simulink model "rfsoc4x2_ospfb_128"  (R2021a)
settings: Solver=VariableStepAuto  StartTime=0.0  StopTime=2048  RelTol=1e-3
undefined symbols (not defined in the file): pfb_coeff_gen_calc
libraries: xbsIndex_r4 x25898, casper_library_delays x113, casper_library_misc x68, xps_library x1
(part 6 of 221)

== system rfsoc4x2_ospfb_128/pipeline ==
  d : Inport
  Register0 : xbsIndex_r4/Register  init=0  rst=off  en=off  dbl_ovrd=off  block_type=register
      settings: block_version=11.4
  Register1 : xbsIndex_r4/Register  init=0  rst=off  en=off  dbl_ovrd=off  block_type=register
  q : Outport  VectorParamsAs1DForOutWhenUnconnected=off
  wires:
  Register0/1 -> Register1/1
  d/1 -> Register0/1
  Register1/1 -> q/1

== system rfsoc4x2_ospfb_128/pipeline1 ==
  d : Inport
  Register0 : xbsIndex_r4/Register  init=0  rst=off  en=off  dbl_ovrd=off  block_type=register
      settings: block_version=11.4
  Register1 : xbsIndex_r4/Register  init=0  rst=off  en=off  dbl_ovrd=off  block_type=register
  q : Outport  VectorParamsAs1DForOutWhenUnconnected=off
  wires:
  Register0/1 -> Register1/1
  d/1 -> Register0/1
  Register1/1 -> q/1

== system rfsoc4x2_ospfb_128/pipeline100 ==
  d : Inport
  Register0 : xbsIndex_r4/Register  init=0  rst=off  en=off  dbl_ovrd=off  block_type=register
      settings: block_version=11.4
  q : Outport  VectorParamsAs1DForOutWhenUnconnected=off
  wires:
  d/1 -> Register0/1
  Register0/1 -> q/1

== system rfsoc4x2_ospfb_128/pipeline101 ==
  d : Inport
  Register0 : xbsIndex_r4/Register  init=0  rst=off  en=off  dbl_ovrd=off  block_type=register
      settings: block_version=11.4
  q : Outport  VectorParamsAs1DForOutWhenUnconnected=off
  wires:
  d/1 -> Register0/1
  Register0/1 -> q/1

== system rfsoc4x2_ospfb_128/pipeline102 ==
  d : Inport
  Register0 : xbsIndex_r4/Register  init=0  rst=off  en=off  dbl_ovrd=off  block_type=register
      settings: block_version=11.4
  q : Outport  VectorParamsAs1DForOutWhenUnconnected=off
  wires:
  d/1 -> Register0/1
  Register0/1 -> q/1

== system rfsoc4x2_ospfb_128/pipeline103 ==
  d : Inport
  Register0 : xbsIndex_r4/Register  init=0  rst=off  en=off  dbl_ovrd=off  block_type=register
      settings: block_version=11.4
  q : Outport  VectorParamsAs1DForOutWhenUnconnected=off
  wires:
  d/1 -> Register0/1
  Register0/1 -> q/1

== system rfsoc4x2_ospfb_128/pipeline104 ==
  d : Inport
  Register0 : xbsIndex_r4/Register  init=0  rst=off  en=off  dbl_ovrd=off  block_type=register
      settings: block_version=11.4
  q : Outport  VectorParamsAs1DForOutWhenUnconnected=off
  wires:
  d/1 -> Register0/1
  Register0/1 -> q/1

== system rfsoc4x2_ospfb_128/pipeline105 ==
  d : Inport
  Register0 : xbsIndex_r4/Register  init=0  rst=off  en=off  dbl_ovrd=off  block_type=register
      settings: block_version=11.4
  q : Outport  VectorParamsAs1DForOutWhenUnconnected=off
  wires:
  d/1 -> Register0/1
  Register0/1 -> q/1

== system rfsoc4x2_ospfb_128/pipeline106 ==
  d : Inport
  Register0 : xbsIndex_r4/Register  init=0  rst=off  en=off  dbl_ovrd=off  block_type=register
      settings: block_version=11.4
  q : Outport  VectorParamsAs1DForOutWhenUnconnected=off
  wires:
  d/1 -> Register0/1
  Register0/1 -> q/1

== system rfsoc4x2_ospfb_128/pipeline2 ==
  d : Inport
  Register0 : xbsIndex_r4/Register  init=0  rst=off  en=off  dbl_ovrd=off  block_type=register
      settings: block_version=11.4
  Register1 : xbsIndex_r4/Register  init=0  rst=off  en=off  dbl_ovrd=off  block_type=register
  q : Outport  VectorParamsAs1DForOutWhenUnconnected=off
  wires:
  Register1/1 -> q/1
  d/1 -> Register0/1
  Register0/1 -> Register1/1

== system rfsoc4x2_ospfb_128/pipeline54 ==
  d : Inport
  Register0 : xbsIndex_r4/Register  init=0  rst=off  en=off  dbl_ovrd=off  block_type=register
      settings: block_version=11.4
  q : Outport  VectorParamsAs1DForOutWhenUnconnected=off
  wires:
  d/1 -> Register0/1
  Register0/1 -> q/1

== system rfsoc4x2_ospfb_128/pipeline55 ==
  d : Inport
  Register0 : xbsIndex_r4/Register  init=0  rst=off  en=off  dbl_ovrd=off  block_type=register
      settings: block_version=11.4
  q : Outport  VectorParamsAs1DForOutWhenUnconnected=off
  wires:
  d/1 -> Register0/1
  Register0/1 -> q/1

== system rfsoc4x2_ospfb_128/pipeline56 ==
  d : Inport
  Register0 : xbsIndex_r4/Register  init=0  rst=off  en=off  dbl_ovrd=off  block_type=register
      settings: block_version=11.4
  q : Outport  VectorParamsAs1DForOutWhenUnconnected=off
  wires:
  d/1 -> Register0/1
  Register0/1 -> q/1

== system rfsoc4x2_ospfb_128/pipeline57 ==
  d : Inport
  Register0 : xbsIndex_r4/Register  init=0  rst=off  en=off  dbl_ovrd=off  block_type=register
      settings: block_version=11.4
  q : Outport  VectorParamsAs1DForOutWhenUnconnected=off
  wires:
  d/1 -> Register0/1
  Register0/1 -> q/1

== system rfsoc4x2_ospfb_128/pipeline58 ==
  d : Inport
  Register0 : xbsIndex_r4/Register  init=0  rst=off  en=off  dbl_ovrd=off  block_type=register
      settings: block_version=11.4
  q : Outport  VectorParamsAs1DForOutWhenUnconnected=off
  wires:
  d/1 -> Register0/1
  Register0/1 -> q/1

== system rfsoc4x2_ospfb_128/pipeline60 ==
  d : Inport
  Register0 : xbsIndex_r4/Register  init=0  rst=off  en=off  dbl_ovrd=off  block_type=register
      settings: block_version=11.4
  q : Outport  VectorParamsAs1DForOutWhenUnconnected=off
  wires:
  d/1 -> Register0/1
  Register0/1 -> q/1

== system rfsoc4x2_ospfb_128/pipeline61 ==
  d : Inport
  Register0 : xbsIndex_r4/Register  init=0  rst=off  en=off  dbl_ovrd=off  block_type=register
      settings: block_version=11.4
  q : Outport  VectorParamsAs1DForOutWhenUnconnected=off
  wires:
  d/1 -> Register0/1
  Register0/1 -> q/1

== system rfsoc4x2_ospfb_128/pipeline62 ==
  d : Inport
  Register0 : xbsIndex_r4/Register  init=0  rst=off  en=off  dbl_ovrd=off  block_type=register
      settings: block_version=11.4
  q : Outport  VectorParamsAs1DForOutWhenUnconnected=off
  wires:
  d/1 -> Register0/1
  Register0/1 -> q/1

== system rfsoc4x2_ospfb_128/pipeline63 ==
  d : Inport
  Register0 : xbsIndex_r4/Register  init=0  rst=off  en=off  dbl_ovrd=off  block_type=register
      settings: block_version=11.4
  q : Outport  VectorParamsAs1DForOutWhenUnconnected=off
  wires:
  d/1 -> Register0/1
  Register0/1 -> q/1

== system rfsoc4x2_ospfb_128/pipeline64 ==
  d : Inport
  Register0 : xbsIndex_r4/Register  init=0  rst=off  en=off  dbl_ovrd=off  block_type=register
      settings: block_version=11.4
  q : Outport  VectorParamsAs1DForOutWhenUnconnected=off
  wires:
  d/1 -> Register0/1
  Register0/1 -> q/1

== system rfsoc4x2_ospfb_128/pipeline65 ==
  d : Inport
  Register0 : xbsIndex_r4/Register  init=0  rst=off  en=off  dbl_ovrd=off  block_type=register
      settings: block_version=11.4
  q : Outport  VectorParamsAs1DForOutWhenUnconnected=off
  wires:
  d/1 -> Register0/1
  Register0/1 -> q/1

== system rfsoc4x2_ospfb_128/pipeline66 ==
  d : Inport
  Register0 : xbsIndex_r4/Register  init=0  rst=off  en=off  dbl_ovrd=off  block_type=register
      settings: block_version=11.4
  q : Outport  VectorParamsAs1DForOutWhenUnconnected=off
  wires:
  d/1 -> Register0/1
  Register0/1 -> q/1

== system rfsoc4x2_ospfb_128/pipeline67 ==
  d : Inport
  Register0 : xbsIndex_r4/Register  init=0  rst=off  en=off  dbl_ovrd=off  block_type=register
      settings: block_version=11.4
  q : Outport  VectorParamsAs1DForOutWhenUnconnected=off
  wires:
  d/1 -> Register0/1
  Register0/1 -> q/1

== system rfsoc4x2_ospfb_128/pipeline68 ==
  d : Inport
  Register0 : xbsIndex_r4/Register  init=0  rst=off  en=off  dbl_ovrd=off  block_type=register
      settings: block_version=11.4
  q : Outport  VectorParamsAs1DForOutWhenUnconnected=off
  wires:
  d/1 -> Register0/1
  Register0/1 -> q/1

== system rfsoc4x2_ospfb_128/pipeline69 ==
  d : Inport
  Register0 : xbsIndex_r4/Register  init=0  rst=off  en=off  dbl_ovrd=off  block_type=register
      settings: block_version=11.4
  q : Outport  VectorParamsAs1DForOutWhenUnconnected=off
  wires:
  d/1 -> Register0/1
  Register0/1 -> q/1

== system rfsoc4x2_ospfb_128/pipeline71 ==
  d : Inport
  Register0 : xbsIndex_r4/Register  init=0  rst=off  en=off  dbl_ovrd=off  block_type=register
      settings: block_version=11.4
  q : Outport  VectorParamsAs1DForOutWhenUnconnected=off
  wires:
  d/1 -> Register0/1
  Register0/1 -> q/1

== system rfsoc4x2_ospfb_128/pipeline72 ==
  d : Inport
  Register0 : xbsIndex_r4/Register  init=0  rst=off  en=off  dbl_ovrd=off  block_type=register
      settings: block_version=11.4
  q : Outport  VectorParamsAs1DForOutWhenUnconnected=off
  wires:
  d/1 -> Register0/1
  Register0/1 -> q/1

== system rfsoc4x2_ospfb_128/pipeline73 ==
  d : Inport
  Register0 : xbsIndex_r4/Register  init=0  rst=off  en=off  dbl_ovrd=off  block_type=register
      settings: block_version=11.4
  q : Outport  VectorParamsAs1DForOutWhenUnconnected=off
  wires:
  d/1 -> Register0/1
  Register0/1 -> q/1

== system rfsoc4x2_ospfb_128/pipeline74 ==
  d : Inport
  Register0 : xbsIndex_r4/Register  init=0  rst=off  en=off  dbl_ovrd=off  block_type=register
      settings: block_version=11.4
  q : Outport  VectorParamsAs1DForOutWhenUnconnected=off
  wires:
  d/1 -> Register0/1
  Register0/1 -> q/1

== system rfsoc4x2_ospfb_128/pipeline75 ==
  d : Inport
  Register0 : xbsIndex_r4/Register  init=0  rst=off  en=off  dbl_ovrd=off  block_type=register
      settings: block_version=11.4
  q : Outport  VectorParamsAs1DForOutWhenUnconnected=off
  wires:
  d/1 -> Register0/1
  Register0/1 -> q/1

== system rfsoc4x2_ospfb_128/pipeline76 ==
  d : Inport
  Register0 : xbsIndex_r4/Register  init=0  rst=off  en=off  dbl_ovrd=off  block_type=register
      settings: block_version=11.4
  q : Outport  VectorParamsAs1DForOutWhenUnconnected=off
  wires:
  d/1 -> Register0/1
  Register0/1 -> q/1

== system rfsoc4x2_ospfb_128/pipeline79 ==
  d : Inport
  Register0 : xbsIndex_r4/Register  init=0  rst=off  en=off  dbl_ovrd=off  block_type=register
      settings: block_version=11.4
  q : Outport  VectorParamsAs1DForOutWhenUnconnected=off
  wires:
  d/1 -> Register0/1
  Register0/1 -> q/1

== system rfsoc4x2_ospfb_128/pipeline80 ==
  d : Inport
  Register0 : xbsIndex_r4/Register  init=0  rst=off  en=off  dbl_ovrd=off  block_type=register
      settings: block_version=11.4
  q : Outport  VectorParamsAs1DForOutWhenUnconnected=off
  wires:
  d/1 -> Register0/1
  Register0/1 -> q/1

== system rfsoc4x2_ospfb_128/pipeline81 ==
  d : Inport
  Register0 : xbsIndex_r4/Register  init=0  rst=off  en=off  dbl_ovrd=off  block_type=register
      settings: block_version=11.4
  q : Outport  VectorParamsAs1DForOutWhenUnconnected=off
  wires:
  d/1 -> Register0/1
  Register0/1 -> q/1

== system rfsoc4x2_ospfb_128/pipeline82 ==
  d : Inport
  Register0 : xbsIndex_r4/Register  init=0  rst=off  en=off  dbl_ovrd=off  block_type=register
      settings: block_version=11.4
  q : Outport  VectorParamsAs1DForOutWhenUnconnected=off
  wires:
  d/1 -> Register0/1
  Register0/1 -> q/1

== system rfsoc4x2_ospfb_128/pipeline83 ==
  d : Inport
  Register0 : xbsIndex_r4/Register  init=0  rst=off  en=off  dbl_ovrd=off  block_type=register
      settings: block_version=11.4
  q : Outport  VectorParamsAs1DForOutWhenUnconnected=off
  wires:
  d/1 -> Register0/1
  Register0/1 -> q/1

== system rfsoc4x2_ospfb_128/pipeline84 ==
  d : Inport
  Register0 : xbsIndex_r4/Register  init=0  rst=off  en=off  dbl_ovrd=off  block_type=register
      settings: block_version=11.4
  q : Outport  VectorParamsAs1DForOutWhenUnconnected=off
  wires:
  d/1 -> Register0/1
  Register0/1 -> q/1

== system rfsoc4x2_ospfb_128/pipeline85 ==
  d : Inport
  Register0 : xbsIndex_r4/Register  init=0  rst=off  en=off  dbl_ovrd=off  block_type=register
      settings: block_version=11.4
  q : Outport  VectorParamsAs1DForOutWhenUnconnected=off
  wires:
  d/1 -> Register0/1
  Register0/1 -> q/1

== system rfsoc4x2_ospfb_128/pipeline86 ==
  d : Inport
  Register0 : xbsIndex_r4/Register  init=0  rst=off  en=off  dbl_ovrd=off  block_type=register
      settings: block_version=11.4
  q : Outport  VectorParamsAs1DForOutWhenUnconnected=off
  wires:
  d/1 -> Register0/1
  Register0/1 -> q/1

== system rfsoc4x2_ospfb_128/pipeline87 ==
  d : Inport
  Register0 : xbsIndex_r4/Register  init=0  rst=off  en=off  dbl_ovrd=off  block_type=register
      settings: block_version=11.4
  q : Outport  VectorParamsAs1DForOutWhenUnconnected=off
  wires:
  d/1 -> Register0/1
  Register0/1 -> q/1

== system rfsoc4x2_ospfb_128/pipeline88 ==
  d : Inport
  Register0 : xbsIndex_r4/Register  init=0  rst=off  en=off  dbl_ovrd=off  block_type=register
      settings: block_version=11.4
  q : Outport  VectorParamsAs1DForOutWhenUnconnected=off
  wires:
  d/1 -> Register0/1
  Register0/1 -> q/1

== system rfsoc4x2_ospfb_128/pipeline89 ==
  d : Inport
  Register0 : xbsIndex_r4/Register  init=0  rst=off  en=off  dbl_ovrd=off  block_type=register
      settings: block_version=11.4
  q : Outport  VectorParamsAs1DForOutWhenUnconnected=off
  wires:
  d/1 -> Register0/1
  Register0/1 -> q/1

== system rfsoc4x2_ospfb_128/pipeline90 ==
  d : Inport
  Register0 : xbsIndex_r4/Register  init=0  rst=off  en=off  dbl_ovrd=off  block_type=register
      settings: block_version=11.4
  q : Outport  VectorParamsAs1DForOutWhenUnconnected=off
  wires:
  d/1 -> Register0/1
  Register0/1 -> q/1

== system rfsoc4x2_ospfb_128/pipeline91 ==
  d : Inport
  Register0 : xbsIndex_r4/Register  init=0  rst=off  en=off  dbl_ovrd=off  block_type=register
      settings: block_version=11.4
  q : Outport  VectorParamsAs1DForOutWhenUnconnected=off
  wires:
  d/1 -> Register0/1
  Register0/1 -> q/1

== system rfsoc4x2_ospfb_128/pipeline92 ==
  d : Inport
  Register0 : xbsIndex_r4/Register  init=0  rst=off  en=off  dbl_ovrd=off  block_type=register
      settings: block_version=11.4
  q : Outport  VectorParamsAs1DForOutWhenUnconnected=off
  wires:
  d/1 -> Register0/1
  Register0/1 -> q/1

== system rfsoc4x2_ospfb_128/pipeline93 ==
  d : Inport
  Register0 : xbsIndex_r4/Register  init=0  rst=off  en=off  dbl_ovrd=off  block_type=register
      settings: block_version=11.4
  q : Outport  VectorParamsAs1DForOutWhenUnconnected=off
  wires:
  d/1 -> Register0/1
  Register0/1 -> q/1

== system rfsoc4x2_ospfb_128/pipeline94 ==
  d : Inport
  Register0 : xbsIndex_r4/Register  init=0  rst=off  en=off  dbl_ovrd=off  block_type=register
      settings: block_version=11.4
  q : Outport  VectorParamsAs1DForOutWhenUnconnected=off
  wires:
  d/1 -> Register0/1
  Register0/1 -> q/1

== system rfsoc4x2_ospfb_128/pipeline95 ==
  d : Inport
  Register0 : xbsIndex_r4/Register  init=0  rst=off  en=off  dbl_ovrd=off  block_type=register
      settings: block_version=11.4
  q : Outport  VectorParamsAs1DForOutWhenUnconnected=off
  wires:
  d/1 -> Register0/1
  Register0/1 -> q/1

== system rfsoc4x2_ospfb_128/pipeline96 ==
  d : Inport
  Register0 : xbsIndex_r4/Register  init=0  rst=off  en=off  dbl_ovrd=off  block_type=register
      settings: block_version=11.4
  q : Outport  VectorParamsAs1DForOutWhenUnconnected=off
  wires:
  d/1 -> Register0/1
  Register0/1 -> q/1

== system rfsoc4x2_ospfb_128/pipeline97 ==
  d : Inport
  Register0 : xbsIndex_r4/Register  init=0  rst=off  en=off  dbl_ovrd=off  block_type=register
      settings: block_version=11.4
  q : Outport  VectorParamsAs1DForOutWhenUnconnected=off
  wires:
  d/1 -> Register0/1
  Register0/1 -> q/1

== system rfsoc4x2_ospfb_128/pipeline98 ==
  d : Inport
  Register0 : xbsIndex_r4/Register  init=0  rst=off  en=off  dbl_ovrd=off  block_type=register
      settings: block_version=11.4
  q : Outport  VectorParamsAs1DForOutWhenUnconnected=off
  wires:
  d/1 -> Register0/1
  Register0/1 -> q/1

== system rfsoc4x2_ospfb_128/pipeline99 ==
  d : Inport
  Register0 : xbsIndex_r4/Register  init=0  rst=off  en=off  dbl_ovrd=off  block_type=register
      settings: block_version=11.4
  q : Outport  VectorParamsAs1DForOutWhenUnconnected=off
  wires:
  d/1 -> Register0/1
  Register0/1 -> q/1
